simulink model "sm_car_Axle3_withDSD"  (R2022a)
settings: Solver=ode23t  StartTime=0.0  StopTime=40  MaxStep=0.4  RelTol=1e-3  AbsTol=1e-3  EnableMultiTasking=on
PreLoadFcn:
  | disp('Loading default data for 3-axle vehicle and 2-axle trailer')
  | if verLessThan('matlab', '9.11')
  |     load Vehicle_Axle3_008
  |     Vehicle = Vehicle_Axle3_008;
  |     load Trailer_Axle2_000
  |     Trailer = Trailer_Axle2_000;
  | else
  |     load Vehicle_Axle3_019
  |     Vehicle = Vehicle_Axle3_019;
  |     load Trailer_Axle2_022
  |     Trailer = Trailer_Axle2_022;
  | end
  | 
  | disp('Turning off MFEval warnings...')
  | disp('Solver:CoeffChecks:Eyk -- OFF')
  | disp('Solver:Limits:Exceeded -- OFF')
  | disp('Solver:CoeffChecks:Et -- OFF')
  | disp('Solver:CoeffChecks:Exa -- OFF')
  | 
  | warning('off','Solver:CoeffChecks:Eyk')
  | warning('off','Solver:Limits:Exceeded')
  | warning('off','Solver:CoeffChecks:Et')
  | warning('off','Solver:CoeffChecks:Exa')
  | %warning('off','Solver:Radius:NegativeRho')
  | 
  | % Due to usability issue in Repeating Sequence block
  | warning('off','Simulink:Masking:Invalid');
  | 
  | % Eliminate unnecessary warnings in inactive variants
  | % Warnings generated only if you click through inactive variant
  | warning('off','MATLAB:nonExistentField');
  | warning('off','Simulink:Parameters:BlkParamUndefined');
PostLoadFcn:
  | set_param([bdroot '/Vehicle'],'popup_trailer','On')
  | warning('off','sm:sli:setup:compile:LocalSolverNotSupported')
  | sm_car_config_maneuver(bdroot,'WOT Braking');
  | sm_car_config_vehicle(bdroot,false);
  | sm_car_config_logging(bdroot);
InitFcn:
  | sm_car_config_camera;
  | Vehicle = sm_car_vehcfg_checkConfig(Vehicle);
StartFcn:
  | sm_car_check_tire_model(bdroot);
  | tic;
StopFcn:
  | Elapsed_Sim_Time = toc;
  | % disp(['Elapsed Sim Time = ' num2str(Elapsed_Sim_Time)]);
values from neighbouring files (symbols this model uses):
  scenario = drivingScenario    [AEB_PedestrianChild_Nearside_50width_overrun.m]
undefined symbols (not defined in the file or in its folder): Maneuver, SimParams, X, Y, Z
libraries: simulink x16, Tire_Utilities x7, sm_lib x6, sm_car_DSD_lib x3, World_Config_Utilities x2, Maneuver_Get_Pose x2, Vehicle_Visualization x2, drivingscenarioandsensors x1, Camera_Frame_Definitions x1, Brake_Control x1, Driveline_Control_Axle2_None x1, Power_Control_Axle2_FixedRatio x1
(part 3 of 3)

== system sm_car_Axle3_withDSD/Visualization/Unreal/Animation On/Unreal Animation ==
  Translation : Inport  OutDataTypeStr=single  PortDimensions=[5,3]
  Rotation : Inport  Port=2  OutDataTypeStr=single  PortDimensions=[5,3]
  Rate Transition1 : RateTransition  Deterministic=off  OutPortSampleTime=0.03
  Rate Transition2 : RateTransition  Deterministic=off  OutPortSampleTime=0.03
  Scale : Subsystem
  Simulation 3D Scene Configuration : sim3dlib/Simulation 3D Scene Configuration  Priority=0  ProjectFormat=Default Scenes  SceneDesc=Double lane change  ProjectName=C:\Program Files\MATLAB\R2022a\toolbox\shared\sim3d_projects\automotive_project\UE4\WindowsNoEditor\VehicleSimulation.exe  ScenePath=/Game/Maps/HwStrght  vehTagList={'Scene Origin';'SimulinkVehicle1'}  vehTag=SimulinkVehicle1  OpVisEn=off  Ts=.03  EnableWindow=on  EnableRemoteAccess=off  EnableWeather=off  SunAltitude=40.0  SunAzimuth=90  clouds=10  wind=1  fog=0  rain=0  sensorTag=MainCamera1  sensorId=1  sensorName=MainCamera1  mountLoc=Origin  offsetFlag=off  tmountOffset=[0, 0, 0]  rmountOffset=[0, 0, 0]  HorizontalResolution=1280  VerticalResolution=720  HorizontalFOV=60  mountPoint=[0 0 0]  mountOrientation=[0 0 0]  aMode=aMode  ID=1
      settings: SourceProductBaseCode=VE,AE,DR,UV,VE
  Simulation 3D Vehicle : sim3dautolib/Simulation 3D Vehicle  Priority=-1  PassVehMesh=Sedan  MeshPath=/MathWorksSimulation/Vehicles/Muscle/Meshes/SK_MuscleCar.SK_MuscleCar  VehColor=Blue  ActorName=SimulinkVehicle1  VehLightsControl=off  HeadlightColor=[ 1, 1, 1 ]  HighBeamIntensity=100000  LowBeamIntensity=60000  HighBeamConeAngle=1.22  LowBeamConeAngle=1.22  LeftHeadlightOrientation=[ 0, 0 ]  RightHeadlightOrientation=[ 0, 0 ]  BrakelightIntensity=500  ReverselightIntensity=500  SignallightIntensity=500  SignallightPeriod=1  SignalPulseWidth=50  Translation=[0 0 1; 0 0 0; 0 0 0; 0 0 0; 0 0 0]  Rotation=[0 0 0; 0 0 0; 0 0 0; 0 0 0; 0 0 0]  Scale=ones( 5, 3 )  SampleTime=.03  ActorType=SimulinkVehicle  ID=1  aMode=2  ActorTag=SimulinkVehicle1
      settings: SourceProductBaseCode=VE,AE,DR,UV,VE
  wires:
  Rotation/1 -> Rate Transition2/1
  Rate Transition1/1 -> Simulation 3D Vehicle/1
  Translation/1 -> Rate Transition1/1
  Rate Transition2/1 -> Simulation 3D Vehicle/2
  Scale/1(ScaleOut) -> Simulation 3D Vehicle/3

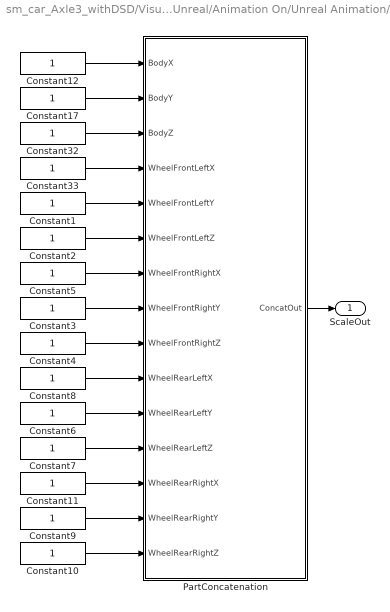
== system sm_car_Axle3_withDSD/Visualization/Unreal/Animation On/Unreal Animation/Scale ==
  Constant{1..12,17,32..33} (15 alike) : Constant  OutDataTypeStr=single
  PartConcatenation : Subsystem
  ScaleOut : Outport  VectorParamsAs1DForOutWhenUnconnected=off
  wires:
  Constant10/1 -> PartConcatenation/15(WheelRearRightZ)
  Constant9/1 -> PartConcatenation/14(WheelRearRightY)
  Constant11/1 -> PartConcatenation/13(WheelRearRightX)
  Constant7/1 -> PartConcatenation/12(WheelRearLeftZ)
  Constant6/1 -> PartConcatenation/11(WheelRearLeftY)
  Constant8/1 -> PartConcatenation/10(WheelRearLeftX)
  Constant4/1 -> PartConcatenation/9(WheelFrontRightZ)
  Constant3/1 -> PartConcatenation/8(WheelFrontRightY)
  Constant5/1 -> PartConcatenation/7(WheelFrontRightX)
  Constant2/1 -> PartConcatenation/6(WheelFrontLeftZ)
  Constant1/1 -> PartConcatenation/5(WheelFrontLeftY)
  Constant33/1 -> PartConcatenation/4(WheelFrontLeftX)
  Constant32/1 -> PartConcatenation/3(BodyZ)
  Constant17/1 -> PartConcatenation/2(BodyY)
  Constant12/1 -> PartConcatenation/1(BodyX)
  PartConcatenation/1(ConcatOut) -> ScaleOut/1

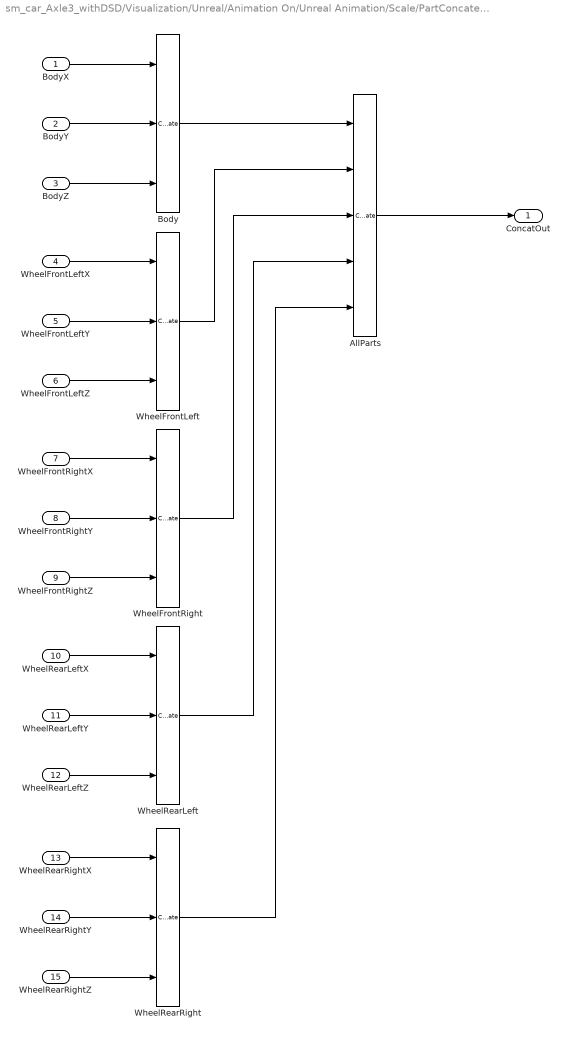
== system sm_car_Axle3_withDSD/Visualization/Unreal/Animation On/Unreal Animation/Scale/PartConcatenation ==
  BodyX : Inport
  BodyY : Inport  Port=2
  BodyZ : Inport  Port=3
  WheelFrontLeftX : Inport  Port=4
  WheelFrontLeftY : Inport  Port=5
  WheelFrontLeftZ : Inport  Port=6
  WheelFrontRightX : Inport  Port=7
  WheelFrontRightY : Inport  Port=8
  WheelFrontRightZ : Inport  Port=9
  WheelRearLeftX : Inport  Port=10
  WheelRearLeftY : Inport  Port=11
  WheelRearLeftZ : Inport  Port=12
  WheelRearRightX : Inport  Port=13
  WheelRearRightY : Inport  Port=14
  WheelRearRightZ : Inport  Port=15
  AllParts : Concatenate  NumInputs=5  Mode=Multidimensional array
  Body : Concatenate  NumInputs=3  Mode=Multidimensional array  ConcatenateDimension=2
  WheelFrontLeft : Concatenate  NumInputs=3  Mode=Multidimensional array  ConcatenateDimension=2
  WheelFrontRight : Concatenate  NumInputs=3  Mode=Multidimensional array  ConcatenateDimension=2
  WheelRearLeft : Concatenate  NumInputs=3  Mode=Multidimensional array  ConcatenateDimension=2
  WheelRearRight : Concatenate  NumInputs=3  Mode=Multidimensional array  ConcatenateDimension=2
  ConcatOut : Outport  VectorParamsAs1DForOutWhenUnconnected=off
  wires:
  BodyX/1 -> Body/1
  BodyZ/1 -> Body/3
  WheelFrontLeftX/1 -> WheelFrontLeft/1
  WheelFrontLeftZ/1 -> WheelFrontLeft/3
  WheelFrontLeftY/1 -> WheelFrontLeft/2
  BodyY/1 -> Body/2
  WheelFrontLeft/1 -> AllParts/2
  WheelRearRightX/1 -> WheelRearRight/1
  Body/1 -> AllParts/1
  WheelRearLeft/1 -> AllParts/4
  WheelFrontRight/1 -> AllParts/3
  WheelRearRightZ/1 -> WheelRearRight/3
  WheelFrontRightY/1 -> WheelFrontRight/2
  WheelFrontRightX/1 -> WheelFrontRight/1
  WheelRearRightY/1 -> WheelRearRight/2
  WheelRearLeftZ/1 -> WheelRearLeft/3
  AllParts/1 -> ConcatOut/1
  WheelRearLeftY/1 -> WheelRearLeft/2
  WheelRearRight/1 -> AllParts/5
  WheelRearLeftX/1 -> WheelRearLeft/1
  WheelFrontRightZ/1 -> WheelFrontRight/3
